simulink model "tb_drive_foc"  (R2026b)
settings: Solver=ode3  StopTime=1  FixedStep=P.drive.Ts_foc_plant  EnableMultiTasking=on
model workspace (MAT data in the model file):
  tb_J = 1.2798
  tb_Rsrc = 0.02
  tb_T_amb = 318.15
  tb_Trr = 6.97491
  tb_cmd.enable = timeseries
  tb_cmd.enable.Name = 'unnamed'
  tb_cmd.enable.DataInfo = tsdata.datametadata
  tb_cmd.enable.DataInfo.Interpolation = tsdata.interpolation
  tb_cmd.enable.DataInfo.Interpolation.Fhandle : function handle (value not decoded)
  tb_cmd.enable.DataInfo.Interpolation.Name = 'linear'
  tb_cmd.enable.TimeInfo = tsdata.timemetadata
  tb_cmd.enable.TimeInfo.Length = 1
  tb_cmd.enable.TimeInfo.DuplicateTimes = 0
  tb_cmd.enable.TimeInfo.Time_ = 0
  tb_cmd.enable.TimeInfo.Initialized = 1
  tb_cmd.enable.QualityInfo = tsdata.qualmetadata
  tb_cmd.enable.Data_ = 0
  tb_cmd.mode = timeseries
  tb_cmd.mode.Name = 'unnamed'
  tb_cmd.mode.DataInfo = tsdata.datametadata
  tb_cmd.mode.DataInfo.Interpolation = tsdata.interpolation
  tb_cmd.mode.DataInfo.Interpolation.Fhandle : function handle (value not decoded)
  tb_cmd.mode.DataInfo.Interpolation.Name = 'linear'
  tb_cmd.mode.TimeInfo = tsdata.timemetadata
  tb_cmd.mode.TimeInfo.Length = 1
  tb_cmd.mode.TimeInfo.DuplicateTimes = 0
  tb_cmd.mode.TimeInfo.Time_ = 0
  tb_cmd.mode.TimeInfo.Initialized = 1
  tb_cmd.mode.QualityInfo = tsdata.qualmetadata
  tb_cmd.mode.Data_ = 1
  tb_cmd.w_ref = timeseries
  tb_cmd.w_ref.Name = 'unnamed'
  tb_cmd.w_ref.DataInfo = tsdata.datametadata
  tb_cmd.w_ref.DataInfo.Interpolation = tsdata.interpolation
  tb_cmd.w_ref.DataInfo.Interpolation.Fhandle : function handle (value not decoded)
  tb_cmd.w_ref.DataInfo.Interpolation.Name = 'linear'
  tb_cmd.w_ref.TimeInfo = tsdata.timemetadata
  tb_cmd.w_ref.TimeInfo.Length = 1
  tb_cmd.w_ref.TimeInfo.DuplicateTimes = 0
  tb_cmd.w_ref.TimeInfo.Time_ = 0
  tb_cmd.w_ref.TimeInfo.Initialized = 1
  tb_cmd.w_ref.QualityInfo = tsdata.qualmetadata
  tb_cmd.w_ref.Data_ = 0
  tb_cmd.tau_ff = timeseries
  tb_cmd.tau_ff.Name = 'unnamed'
  tb_cmd.tau_ff.DataInfo = tsdata.datametadata
  tb_cmd.tau_ff.DataInfo.Interpolation = tsdata.interpolation
  tb_cmd.tau_ff.DataInfo.Interpolation.Fhandle : function handle (value not decoded)
  tb_cmd.tau_ff.DataInfo.Interpolation.Name = 'linear'
  tb_cmd.tau_ff.TimeInfo = tsdata.timemetadata
  tb_cmd.tau_ff.TimeInfo.Length = 1
  tb_cmd.tau_ff.TimeInfo.DuplicateTimes = 0
  tb_cmd.tau_ff.TimeInfo.Time_ = 0
  tb_cmd.tau_ff.TimeInfo.Initialized = 1
  tb_cmd.tau_ff.QualityInfo = tsdata.qualmetadata
  tb_cmd.tau_ff.Data_ = 0
  tb_cmd.tau_lim_mot = timeseries
  tb_cmd.tau_lim_mot.Name = 'unnamed'
  tb_cmd.tau_lim_mot.DataInfo = tsdata.datametadata
  tb_cmd.tau_lim_mot.DataInfo.Interpolation = tsdata.interpolation
  tb_cmd.tau_lim_mot.DataInfo.Interpolation.Fhandle : function handle (value not decoded)
  tb_cmd.tau_lim_mot.DataInfo.Interpolation.Name = 'linear'
  tb_cmd.tau_lim_mot.TimeInfo = tsdata.timemetadata
  tb_cmd.tau_lim_mot.TimeInfo.Length = 1
  tb_cmd.tau_lim_mot.TimeInfo.DuplicateTimes = 0
  tb_cmd.tau_lim_mot.TimeInfo.Time_ = 0
  tb_cmd.tau_lim_mot.TimeInfo.Initialized = 1
  tb_cmd.tau_lim_mot.QualityInfo = tsdata.qualmetadata
  tb_cmd.tau_lim_mot.Data_ = 16
  tb_cmd.tau_lim_reg = timeseries
  tb_cmd.tau_lim_reg.Name = 'unnamed'
  tb_cmd.tau_lim_reg.DataInfo = tsdata.datametadata
  tb_cmd.tau_lim_reg.DataInfo.Interpolation = tsdata.interpolation
  tb_cmd.tau_lim_reg.DataInfo.Interpolation.Fhandle : function handle (value not decoded)
  tb_cmd.tau_lim_reg.DataInfo.Interpolation.Name = 'linear'
  tb_cmd.tau_lim_reg.TimeInfo = tsdata.timemetadata
  tb_cmd.tau_lim_reg.TimeInfo.Length = 1
  tb_cmd.tau_lim_reg.TimeInfo.DuplicateTimes = 0
  tb_cmd.tau_lim_reg.TimeInfo.Time_ = 0
  tb_cmd.tau_lim_reg.TimeInfo.Initialized = 1
  tb_cmd.tau_lim_reg.QualityInfo = tsdata.qualmetadata
  tb_cmd.tau_lim_reg.Data_ = 16
  tb_cmd.park_req = timeseries
  tb_cmd.park_req.Name = 'unnamed'
  tb_cmd.park_req.DataInfo = tsdata.datametadata
  tb_cmd.park_req.DataInfo.Interpolation = tsdata.interpolation
  tb_cmd.park_req.DataInfo.Interpolation.Fhandle : function handle (value not decoded)
  tb_cmd.park_req.DataInfo.Interpolation.Name = 'linear'
  tb_cmd.park_req.TimeInfo = tsdata.timemetadata
  tb_cmd.park_req.TimeInfo.Length = 1
  tb_cmd.park_req.TimeInfo.DuplicateTimes = 0
  tb_cmd.park_req.TimeInfo.Time_ = 0
  tb_cmd.park_req.TimeInfo.Initialized = 1
  tb_cmd.park_req.QualityInfo = tsdata.qualmetadata
  tb_cmd.park_req.Data_ = 0
  tb_cmd.fault_reset = timeseries
  tb_cmd.fault_reset.Name = 'unnamed'
  tb_cmd.fault_reset.DataInfo = tsdata.datametadata
  tb_cmd.fault_reset.DataInfo.Interpolation = tsdata.interpolation
  tb_cmd.fault_reset.DataInfo.Interpolation.Fhandle : function handle (value not decoded)
  tb_cmd.fault_reset.DataInfo.Interpolation.Name = 'linear'
  tb_cmd.fault_reset.TimeInfo = tsdata.timemetadata
  tb_cmd.fault_reset.TimeInfo.Length = 1
  tb_cmd.fault_reset.TimeInfo.DuplicateTimes = 0
  tb_cmd.fault_reset.TimeInfo.Time_ = 0
  tb_cmd.fault_reset.TimeInfo.Initialized = 1
  tb_cmd.fault_reset.QualityInfo = tsdata.qualmetadata
  tb_cmd.fault_reset.Data_ = 0
  tb_cmd.alive = timeseries
  tb_cmd.alive.Name = 'unnamed'
  tb_cmd.alive.DataInfo = tsdata.datametadata
  tb_cmd.alive.DataInfo.Interpolation = tsdata.interpolation
  tb_cmd.alive.DataInfo.Interpolation.Fhandle : function handle (value not decoded)
  tb_cmd.alive.DataInfo.Interpolation.Name = 'linear'
  tb_cmd.alive.TimeInfo = tsdata.timemetadata
  tb_cmd.alive.TimeInfo.Length = 1
  tb_cmd.alive.TimeInfo.DuplicateTimes = 0
  tb_cmd.alive.TimeInfo.Time_ = 0
  tb_cmd.alive.TimeInfo.Initialized = 1
  tb_cmd.alive.QualityInfo = tsdata.qualmetadata
  tb_cmd.alive.Data_ = 0
  tb_contactor = timeseries
  tb_contactor.Name = 'unnamed'
  tb_contactor.DataInfo = tsdata.datametadata
  tb_contactor.DataInfo.Interpolation = tsdata.interpolation
  tb_contactor.DataInfo.Interpolation.Fhandle : function handle (value not decoded)
  tb_contactor.DataInfo.Interpolation.Name = 'linear'
  tb_contactor.TimeInfo = tsdata.timemetadata
  tb_contactor.TimeInfo.Length = 1
  tb_contactor.TimeInfo.DuplicateTimes = 0
  tb_contactor.TimeInfo.Time_ = 0
  tb_contactor.TimeInfo.Initialized = 1
  tb_contactor.QualityInfo = tsdata.qualmetadata
  tb_contactor.Data_ = 1
  tb_dec = 1
  tb_drop = timeseries
  tb_drop.Name = 'unnamed'
  tb_drop.DataInfo = tsdata.datametadata
  tb_drop.DataInfo.Interpolation = tsdata.interpolation
  tb_drop.DataInfo.Interpolation.Fhandle : function handle (value not decoded)
  tb_drop.DataInfo.Interpolation.Name = 'linear'
  tb_drop.TimeInfo = tsdata.timemetadata
  tb_drop.TimeInfo.Length = 1
  tb_drop.TimeInfo.DuplicateTimes = 0
  tb_drop.TimeInfo.Time_ = 0
  tb_drop.TimeInfo.Initialized = 1
  tb_drop.QualityInfo = tsdata.qualmetadata
  tb_drop.Data_ = 0
  tb_fi.L.can_drop = timeseries
  tb_fi.L.can_drop.Name = 'unnamed'
  tb_fi.L.can_drop.DataInfo = tsdata.datametadata
  tb_fi.L.can_drop.DataInfo.Interpolation = tsdata.interpolation
  tb_fi.L.can_drop.DataInfo.Interpolation.Fhandle : function handle (value not decoded)
  tb_fi.L.can_drop.DataInfo.Interpolation.Name = 'linear'
  tb_fi.L.can_drop.TimeInfo = tsdata.timemetadata
  tb_fi.L.can_drop.TimeInfo.Length = 1
  tb_fi.L.can_drop.TimeInfo.DuplicateTimes = 0
  tb_fi.L.can_drop.TimeInfo.Time_ = 0
  tb_fi.L.can_drop.TimeInfo.Initialized = 1
  tb_fi.L.can_drop.QualityInfo = tsdata.qualmetadata
  tb_fi.L.can_drop.Data_ = 0
  tb_fi.L.enc_fail = timeseries
  tb_fi.L.enc_fail.Name = 'unnamed'
  tb_fi.L.enc_fail.DataInfo = tsdata.datametadata
  tb_fi.L.enc_fail.DataInfo.Interpolation = tsdata.interpolation
  tb_fi.L.enc_fail.DataInfo.Interpolation.Fhandle : function handle (value not decoded)
  tb_fi.L.enc_fail.DataInfo.Interpolation.Name = 'linear'
  tb_fi.L.enc_fail.TimeInfo = tsdata.timemetadata
  tb_fi.L.enc_fail.TimeInfo.Length = 1
  tb_fi.L.enc_fail.TimeInfo.DuplicateTimes = 0
  tb_fi.L.enc_fail.TimeInfo.Time_ = 0
  tb_fi.L.enc_fail.TimeInfo.Initialized = 1
  tb_fi.L.enc_fail.QualityInfo = tsdata.qualmetadata
  tb_fi.L.enc_fail.Data_ = 0
  tb_fi.L.brake_stuck = timeseries
  tb_fi.L.brake_stuck.Name = 'unnamed'
  tb_fi.L.brake_stuck.DataInfo = tsdata.datametadata
  tb_fi.L.brake_stuck.DataInfo.Interpolation = tsdata.interpolation
  tb_fi.L.brake_stuck.DataInfo.Interpolation.Fhandle : function handle (value not decoded)
  tb_fi.L.brake_stuck.DataInfo.Interpolation.Name = 'linear'
  tb_fi.L.brake_stuck.TimeInfo = tsdata.timemetadata
  tb_fi.L.brake_stuck.TimeInfo.Length = 1
  tb_fi.L.brake_stuck.TimeInfo.DuplicateTimes = 0
  tb_fi.L.brake_stuck.TimeInfo.Time_ = 0
  tb_fi.L.brake_stuck.TimeInfo.Initialized = 1
  tb_fi.L.brake_stuck.QualityInfo = tsdata.qualmetadata
  tb_fi.L.brake_stuck.Data_ = 0
  tb_fi.L.tau_scale = timeseries
  tb_fi.L.tau_scale.Name = 'unnamed'
  tb_fi.L.tau_scale.DataInfo = tsdata.datametadata
  tb_fi.L.tau_scale.DataInfo.Interpolation = tsdata.interpolation
  tb_fi.L.tau_scale.DataInfo.Interpolation.Fhandle : function handle (value not decoded)
  tb_fi.L.tau_scale.DataInfo.Interpolation.Name = 'linear'
  tb_fi.L.tau_scale.TimeInfo = tsdata.timemetadata
  tb_fi.L.tau_scale.TimeInfo.Length = 1
  tb_fi.L.tau_scale.TimeInfo.DuplicateTimes = 0
  tb_fi.L.tau_scale.TimeInfo.Time_ = 0
  tb_fi.L.tau_scale.TimeInfo.Initialized = 1
  tb_fi.L.tau_scale.QualityInfo = tsdata.qualmetadata
  tb_fi.L.tau_scale.Data_ = 1
  tb_fi.L.T_offset = timeseries
  tb_fi.L.T_offset.Name = 'unnamed'
  tb_fi.L.T_offset.DataInfo = tsdata.datametadata
  tb_fi.L.T_offset.DataInfo.Interpolation = tsdata.interpolation
  tb_fi.L.T_offset.DataInfo.Interpolation.Fhandle : function handle (value not decoded)
  tb_fi.L.T_offset.DataInfo.Interpolation.Name = 'linear'
  tb_fi.L.T_offset.TimeInfo = tsdata.timemetadata
  tb_fi.L.T_offset.TimeInfo.Length = 1
  tb_fi.L.T_offset.TimeInfo.DuplicateTimes = 0
  tb_fi.L.T_offset.TimeInfo.Time_ = 0
  tb_fi.L.T_offset.TimeInfo.Initialized = 1
  tb_fi.L.T_offset.QualityInfo = tsdata.qualmetadata
  tb_fi.L.T_offset.Data_ = 0
  tb_fi.R.can_drop = timeseries
  tb_fi.R.can_drop.Name = 'unnamed'
  tb_fi.R.can_drop.DataInfo = tsdata.datametadata
  tb_fi.R.can_drop.DataInfo.Interpolation = tsdata.interpolation
  tb_fi.R.can_drop.DataInfo.Interpolation.Fhandle : function handle (value not decoded)
  tb_fi.R.can_drop.DataInfo.Interpolation.Name = 'linear'
  tb_fi.R.can_drop.TimeInfo = tsdata.timemetadata
  tb_fi.R.can_drop.TimeInfo.Length = 1
  tb_fi.R.can_drop.TimeInfo.DuplicateTimes = 0
  tb_fi.R.can_drop.TimeInfo.Time_ = 0
  tb_fi.R.can_drop.TimeInfo.Initialized = 1
  tb_fi.R.can_drop.QualityInfo = tsdata.qualmetadata
  tb_fi.R.can_drop.Data_ = 0
  tb_fi.R.enc_fail = timeseries
  tb_fi.R.enc_fail.Name = 'unnamed'
  tb_fi.R.enc_fail.DataInfo = tsdata.datametadata
  tb_fi.R.enc_fail.DataInfo.Interpolation = tsdata.interpolation
  tb_fi.R.enc_fail.DataInfo.Interpolation.Fhandle : function handle (value not decoded)
  tb_fi.R.enc_fail.DataInfo.Interpolation.Name = 'linear'
  tb_fi.R.enc_fail.TimeInfo = tsdata.timemetadata
  tb_fi.R.enc_fail.TimeInfo.Length = 1
  tb_fi.R.enc_fail.TimeInfo.DuplicateTimes = 0
  tb_fi.R.enc_fail.TimeInfo.Time_ = 0
  tb_fi.R.enc_fail.TimeInfo.Initialized = 1
  tb_fi.R.enc_fail.QualityInfo = tsdata.qualmetadata
  tb_fi.R.enc_fail.Data_ = 0
  tb_fi.R.brake_stuck = timeseries
  tb_fi.R.brake_stuck.Name = 'unnamed'
  tb_fi.R.brake_stuck.DataInfo = tsdata.datametadata
  tb_fi.R.brake_stuck.DataInfo.Interpolation = tsdata.interpolation
  tb_fi.R.brake_stuck.DataInfo.Interpolation.Fhandle : function handle (value not decoded)
  tb_fi.R.brake_stuck.DataInfo.Interpolation.Name = 'linear'
  tb_fi.R.brake_stuck.TimeInfo = tsdata.timemetadata
  tb_fi.R.brake_stuck.TimeInfo.Length = 1
  tb_fi.R.brake_stuck.TimeInfo.DuplicateTimes = 0
  tb_fi.R.brake_stuck.TimeInfo.Time_ = 0
  tb_fi.R.brake_stuck.TimeInfo.Initialized = 1
  tb_fi.R.brake_stuck.QualityInfo = tsdata.qualmetadata
  tb_fi.R.brake_stuck.Data_ = 0
  tb_fi.R.tau_scale = timeseries
  tb_fi.R.tau_scale.Name = 'unnamed'
  tb_fi.R.tau_scale.DataInfo = tsdata.datametadata
  tb_fi.R.tau_scale.DataInfo.Interpolation = tsdata.interpolation
  tb_fi.R.tau_scale.DataInfo.Interpolation.Fhandle : function handle (value not decoded)
  tb_fi.R.tau_scale.DataInfo.Interpolation.Name = 'linear'
  tb_fi.R.tau_scale.TimeInfo = tsdata.timemetadata
  tb_fi.R.tau_scale.TimeInfo.Length = 1
  tb_fi.R.tau_scale.TimeInfo.DuplicateTimes = 0
  tb_fi.R.tau_scale.TimeInfo.Time_ = 0
  tb_fi.R.tau_scale.TimeInfo.Initialized = 1
  tb_fi.R.tau_scale.QualityInfo = tsdata.qualmetadata
  tb_fi.R.tau_scale.Data_ = 1
  tb_fi.R.T_offset = timeseries
  tb_fi.R.T_offset.Name = 'unnamed'
  tb_fi.R.T_offset.DataInfo = tsdata.datametadata
  tb_fi.R.T_offset.DataInfo.Interpolation = tsdata.interpolation
  tb_fi.R.T_offset.DataInfo.Interpolation.Fhandle : function handle (value not decoded)
  tb_fi.R.T_offset.DataInfo.Interpolation.Name = 'linear'
  tb_fi.R.T_offset.TimeInfo = tsdata.timemetadata
  tb_fi.R.T_offset.TimeInfo.Length = 1
  tb_fi.R.T_offset.TimeInfo.DuplicateTimes = 0
  tb_fi.R.T_offset.TimeInfo.Time_ = 0
  tb_fi.R.T_offset.TimeInfo.Initialized = 1
  tb_fi.R.T_offset.QualityInfo = tsdata.qualmetadata
  tb_fi.R.T_offset.Data_ = 0
  tb_grade = timeseries
  tb_grade.Name = 'unnamed'
  tb_grade.DataInfo = tsdata.datametadata
  tb_grade.DataInfo.Interpolation = tsdata.interpolation
  tb_grade.DataInfo.Interpolation.Fhandle : function handle (value not decoded)
  tb_grade.DataInfo.Interpolation.Name = 'linear'
  tb_grade.TimeInfo = tsdata.timemetadata
  tb_grade.TimeInfo.Length = 1
  tb_grade.TimeInfo.DuplicateTimes = 0
  tb_grade.TimeInfo.Time_ = 0
  tb_grade.TimeInfo.Initialized = 1
  tb_grade.QualityInfo = tsdata.qualmetadata
  tb_grade.Data_ = 0
  tb_load = 1
  tb_sto = timeseries
  tb_sto.Name = 'unnamed'
  tb_sto.DataInfo = tsdata.datametadata
  tb_sto.DataInfo.Interpolation = tsdata.interpolation
  tb_sto.DataInfo.Interpolation.Fhandle : function handle (value not decoded)
  tb_sto.DataInfo.Interpolation.Name = 'linear'
  tb_sto.TimeInfo = tsdata.timemetadata
  tb_sto.TimeInfo.Length = 1
  tb_sto.TimeInfo.DuplicateTimes = 0
  tb_sto.TimeInfo.Time_ = 0
  tb_sto.TimeInfo.Initialized = 1
  tb_sto.QualityInfo = tsdata.qualmetadata
  tb_sto.Data_ = 1
  tb_vsrc = timeseries
  tb_vsrc.Name = 'unnamed'
  tb_vsrc.DataInfo = tsdata.datametadata
  tb_vsrc.DataInfo.Interpolation = tsdata.interpolation
  tb_vsrc.DataInfo.Interpolation.Fhandle : function handle (value not decoded)
  tb_vsrc.DataInfo.Interpolation.Name = 'linear'
  tb_vsrc.TimeInfo = tsdata.timemetadata
  tb_vsrc.TimeInfo.Length = 1
  tb_vsrc.TimeInfo.DuplicateTimes = 0
  tb_vsrc.TimeInfo.Time_ = 0
  tb_vsrc.TimeInfo.Initialized = 1
  tb_vsrc.QualityInfo = tsdata.qualmetadata
  tb_vsrc.Data_ = 46.8
  tb_w_dyno = timeseries
  tb_w_dyno.Name = 'unnamed'
  tb_w_dyno.DataInfo = tsdata.datametadata
  tb_w_dyno.DataInfo.Interpolation = tsdata.interpolation
  tb_w_dyno.DataInfo.Interpolation.Fhandle : function handle (value not decoded)
  tb_w_dyno.DataInfo.Interpolation.Name = 'linear'
  tb_w_dyno.TimeInfo = tsdata.timemetadata
  tb_w_dyno.TimeInfo.Length = 1
  tb_w_dyno.TimeInfo.DuplicateTimes = 0
  tb_w_dyno.TimeInfo.Time_ = 0
  tb_w_dyno.TimeInfo.Initialized = 1
  tb_w_dyno.QualityInfo = tsdata.qualmetadata
  tb_w_dyno.Data_ = 0
values from neighbouring files (symbols this model uses):
  P = evalin('base', 'P')    [build_tb_drive.m]    (also in tb_drive_long.m; tb_drive_profile.m)
undefined symbols (not defined in the file or in its folder): DiscIntNeverNeededParam
libraries: fl_lib x10, nesl_utility x5, simulink x1
settings Model: Creator=aomar  LastModifiedBy=aomar
settings ConfigSet: Description=Shaddad fixed-step 1 ms ode3, multitasking, explicit rate transitions (arch 7, D58).
settings DataIOCC: SignalLogging=off
settings OptimizationCC: SimCompilerOptimization=on
settings DebuggingCC: AlgebraicLoopMsg=error  ArtificialAlgebraicLoopMsg=error  SingleTaskRateTransMsg=error  StrictBusMsg=ErrorOnBusTreatedAsVector
settings SimscapeCC: SimscapeNominalValues="[{\"value\":\"1\",\"unit\":\"A\"},{\"value\":\"1\",\"unit\":\"bar\"},{\"value\":\"1\",\"unit\":\"cm^2\"},{\"value\":\"1\",\"unit\":\"cm^3/s\"},{\"value\":\"1\",\"unit\":\"kJ/kg\"},{\"value\":\"1\",\"unit\":\"kW\"},{\"value\":\"1\",\"unit\":\"l\"},{\"value\":\"1\",\"unit\":\"N\"},{\"value\":\"1\",\"unit\":\"N*m\"},{\"value\":\"1\",\"unit\":\"V\"},{\"value\":\"0.001\",\"unit\":\"Wb\"}]"  SimscapeNormalizeSystem=off  SimscapeUseEnergyAccounting=off

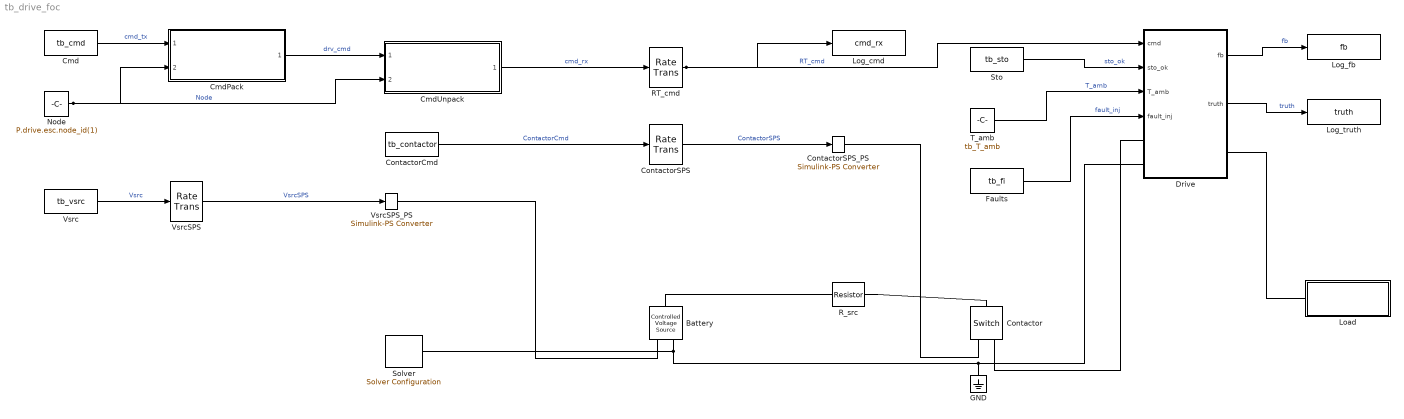
== system tb_drive_foc ==
  Battery : fl_lib/Electrical/Electrical Sources/Controlled Voltage Source
  Cmd : FromWorkspace  VariableName=tb_cmd  OutDataTypeStr=Bus: Bus_DriveSideCmd  SampleTime=P.drive.Ts_can  Interpolate=off  OutputAfterFinalValue=Holding final value
  CmdPack : Subsystem  ReferencedSubsystem=drive_cmd_pack
  CmdUnpack : Subsystem  ReferencedSubsystem=drive_cmd_unpack
  Contactor : fl_lib/Electrical/Electrical Elements/Switch  R_closed=1e-4 Ohm  G_open=1e-8 1/Ohm  Threshold=0.5  i_specify=off  i_priority=None  i=0 A  i_nominal_specify=off  i_nominal_value=1  i_nominal_unit=A  v_specify=off  v_priority=None  v=0 V  v_nominal_specify=off  v_nominal_value=1  v_nominal_unit=V
  ContactorCmd : FromWorkspace  VariableName=tb_contactor  SampleTime=P.drive.Ts_esc  Interpolate=off  OutputAfterFinalValue=Holding final value
  ContactorSPS : RateTransition  OutPortSampleTimeOpt=Inherit
  ContactorSPS_PS : nesl_utility/Simulink-PS Converter  PhysicalDomain=network_engine_domain  SubClassName=ps_input  LeftPortType=input  RightPortType=output  PseudoPeriodic=off  Frequencies=[]  NoiseDistribution=none  NoiseParameters=[]  Unit=1  AffineConversion=off  FilteringAndDerivatives=zero  SimscapeFilterOrder=1  InputFilterTimeConstant=0.001  UdotUserProvided=0
  Drive : Subsystem  mask{side=1}
  Faults : FromWorkspace  VariableName=tb_fi  OutDataTypeStr=Bus: Bus_DriveFaultInj  SampleTime=P.drive.Ts_esc  Interpolate=off  OutputAfterFinalValue=Holding final value
  GND : fl_lib/Electrical/Electrical Elements/Electrical Reference
  Load : Subsystem  Variant=on
  Log_cmd : ToWorkspace  VariableName=cmd_rx  SaveFormat=Timeseries  SampleTime=-1
      settings: Decimation=tb_dec
  Log_fb : ToWorkspace  VariableName=fb  SaveFormat=Timeseries  SampleTime=-1
      settings: Decimation=tb_dec
  Log_truth : ToWorkspace  VariableName=truth  SaveFormat=Timeseries  SampleTime=-1
      settings: Decimation=tb_dec
  Node : Constant  Value=P.drive.esc.node_id(1)  OutDataTypeStr=uint8
  RT_cmd : RateTransition  OutPortSampleTime=P.drive.Ts_esc
  R_src : fl_lib/Electrical/Electrical Elements/Resistor  R=tb_Rsrc Ohm  i_specify=off  i_priority=None  i=0 A  i_nominal_specify=off  i_nominal_value=1  i_nominal_unit=A  v_specify=off  v_priority=None  v=0 V  v_nominal_specify=off  v_nominal_value=1  v_nominal_unit=V
  Solver : nesl_utility/Solver Configuration  PhysicalDomain=network_engine_domain  SubClassName=solver  LeftPortType=input  RightPortType=generic  Tones=[]  Harmonics=[]  SimulateNoise=off  Profile=off  UseLocalSampling=off  EnableSwitchedLinearOptims=on  FrequencyDomain=off  UseCCode=off  RelTol=0.001  AbsTol=0.001  MinStep=1e-09  ToWorkspace=off  RevertToSquareIcSolve=off  NumHomotopyIterations=100  PhasorMode=off  PhasorModeNumHarmonics=1  ConsistencySolver=NEWTON_XTOL_AFTER_FTOL  CanonicalOrdering=CANONICAL  OptimizeIntermediates=OPTIMIZED  MulticoreSolverChoice=BACKWARD_EULER  IndexReductionMethod=DerivativeReplacement  DoDC=off  ResidualTolerance=1e-09  ConsistencyTolSource=GLOBAL  ConsistencyAbsTol=0.001  ConsistencyRelTol=0.001  ConsistencyTolFactor=0.001  UseLocalSolver=on  LocalSolverChoice=NE_BACKWARD_EULER_ADVANCER  ResolveIndetEquations=on  FunctionEvalNumThread=1  LocalSolverSampleTime=P.drive.Ts_foc_plant  DoFixedCost=on  MaxNonlinIter=P.sim.ssc.MaxNonlinIter  MaxModeIter=P.sim.ssc.MaxModeIter  ComputeImpulses=off  ImpulseIterations=2  LinearAlgebra=auto  LinearAlgebraNumThread=0  EquationFormulation=NE_TIME_EF  DelaysMemoryBudget=1024  AutomaticFiltering=on  FilteringTimeConstant=0.001  PartitionStorageMethod=AS_NEEDED  PartitionMemoryBudget=1024  PartitionMethod=BALANCED  MultibodyUseLocalSolver=off  MultibodyLocalSolverChoice=ODE1  MultibodyLocalSolverSampleTime=0.001
  Sto : FromWorkspace  VariableName=tb_sto  OutDataTypeStr=boolean  SampleTime=P.drive.Ts_esc  Interpolate=off  OutputAfterFinalValue=Holding final value
  T_amb : Constant  Value=tb_T_amb  SampleTime=P.drive.Ts_esc
  Vsrc : FromWorkspace  VariableName=tb_vsrc  SampleTime=P.drive.Ts_esc  Interpolate=off  OutputAfterFinalValue=Holding final value
  VsrcSPS : RateTransition  OutPortSampleTimeOpt=Inherit
  VsrcSPS_PS : nesl_utility/Simulink-PS Converter  PhysicalDomain=network_engine_domain  SubClassName=ps_input  LeftPortType=input  RightPortType=output  PseudoPeriodic=off  Frequencies=[]  NoiseDistribution=none  NoiseParameters=[]  Unit=V  AffineConversion=off  FilteringAndDerivatives=zero  SimscapeFilterOrder=1  InputFilterTimeConstant=0.001  UdotUserProvided=0
  wires:
  Node/1 -> CmdPack/2, CmdUnpack/2  "Node"
  Cmd/1 -> CmdPack/1  "cmd_tx"
  Vsrc/1 -> VsrcSPS/1  "Vsrc"
  VsrcSPS/1 -> VsrcSPS_PS/1  "VsrcSPS"
  CmdPack/1 -> CmdUnpack/1  "drv_cmd"
  ContactorCmd/1 -> ContactorSPS/1  "ContactorCmd"
  CmdUnpack/1 -> RT_cmd/1  "cmd_rx"
  RT_cmd/1 -> Log_cmd/1, Drive/1(cmd)  "RT_cmd"
  ContactorSPS/1 -> ContactorSPS_PS/1  "ContactorSPS"
  T_amb/1 -> Drive/3(T_amb)  "T_amb"
  Sto/1 -> Drive/2(sto_ok)  "sto_ok"
  Faults/1 -> Drive/4(fault_inj)  "fault_inj"
  Drive/1(fb) -> Log_fb/1  "fb"
  Drive/2(truth) -> Log_truth/1  "truth"
  connections:
  Battery/LConn1 -- R_src/LConn1
  VsrcSPS_PS/RConn1 -- Battery/RConn1
  R_src/RConn1 -- Contactor/LConn1
  Drive/LConn1 -- Contactor/RConn2
  Drive/RConn1 -- Load/LConn1
  Battery/RConn2 -- Solver/RConn1 -- GND/LConn1 -- Drive/LConn2
  ContactorSPS_PS/RConn1 -- Contactor/RConn1

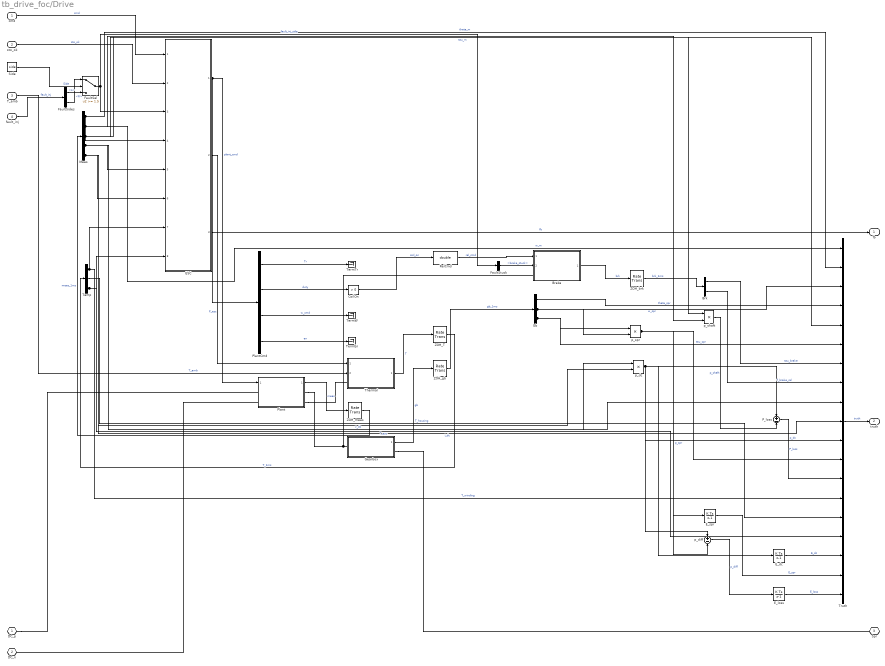
== system tb_drive_foc/Drive ==
  cmd : Inport  OutDataTypeStr=Bus: Bus_DriveSideCmd  SampleTime=P.drive.Ts_esc
  sto_ok : Inport  Port=2  OutDataTypeStr=boolean  SampleTime=P.drive.Ts_esc
  T_amb : Inport  Port=3  OutDataTypeStr=double  SampleTime=P.drive.Ts_esc
  fault_inj : Inport  Port=4  OutDataTypeStr=Bus: Bus_DriveFaultInj  SampleTime=P.drive.Ts_esc
  Brake : Subsystem  ReferencedSubsystem=drive_brake
  Brk : Demux  Outputs=2
  CoilOn : simulink/Logic and Bit Operations/Compare To Constant  relop=>  const=0  OutDataTypeStr=boolean
  ESC : Subsystem  ReferencedSubsystem=drive_esc
  E_dc : DiscreteIntegrator  gainval=1  SampleTime=P.drive.Ts_esc  ICPrevOutput=DiscIntNeverNeededParam  ICPrevScaledInput=DiscIntNeverNeededParam
  E_loss : DiscreteIntegrator  gainval=1  SampleTime=P.drive.Ts_esc  ICPrevOutput=DiscIntNeverNeededParam  ICPrevScaledInput=DiscIntNeverNeededParam
  E_spr : DiscreteIntegrator  gainval=1  SampleTime=P.drive.Ts_esc  ICPrevOutput=DiscIntNeverNeededParam  ICPrevScaledInput=DiscIntNeverNeededParam
  FaultSel : Switch  Threshold=1.5  SaturateOnIntegerOverflow=off  InputSameDT=off
  FaultSides : BusSelector  OutputSignals=L,R
  FaultStuck : BusSelector  OutputSignals=brake_stuck
  Gb : Demux  Outputs=3
  Gearbox : Subsystem  ReferencedSubsystem=drive_gearbox
  Meas : Demux  Outputs=5
  P_loss : Sum  Inputs=+-
  Plant : Subsystem  ReferencedSubsystem=drive_plant_foc
  PlantCmd : Demux
  RelCmd : DataTypeConversion  OutDataTypeStr=double  RndMeth=Nearest
  Side : Constant  Value=side
  Temp : Demux  Outputs=3
  TermEn : Terminator
  TermTr : Terminator
  TermW : Terminator
  Thermal : Subsystem  ReferencedSubsystem=drive_thermal
  Truth : BusCreator  Inputs=19  OutDataTypeStr=Bus: Bus_DriveSideTruth  NonVirtualBus=on
  ZOH_T : RateTransition  OutPortSampleTime=P.drive.Ts_esc
  ZOH_brk : RateTransition  OutPortSampleTime=P.drive.Ts_esc
  ZOH_gb : RateTransition  OutPortSampleTime=P.drive.Ts_esc
  ZOH_meas : RateTransition  OutPortSampleTime=P.drive.Ts_esc
  p_dc : Product  Inputs=**
  p_diff : Sum  Inputs=+-
  p_shaft : Product  Inputs=**
  p_spr : Product  Inputs=**
  DC_p : PMIOPort  Side=Left  ConnectionType=Connection: foundation.electrical.electrical
  DC_n : PMIOPort  Port=2  Side=Left  ConnectionType=Connection: foundation.electrical.electrical
  Spr : PMIOPort  Port=3  Side=Right  ConnectionType=Connection: foundation.mechanical.rotational.rotational
  fb : Outport  OutDataTypeStr=Bus: Bus_DriveSideFb
  truth : Outport  Port=2  OutDataTypeStr=Bus: Bus_DriveSideTruth
  wires:
  cmd/1 -> ESC/1  "cmd"
  sto_ok/1 -> ESC/2  "sto_ok"
  Side/1 -> FaultSel/2  "Side"
  T_amb/1 -> Thermal/2  "T_amb"
  fault_inj/1 -> FaultSides/1  "fault_inj"
  FaultSides/1 -> FaultSel/3  "<L>"
  FaultSides/2 -> FaultSel/1  "<R>"
  Meas/1 -> Truth/2, ESC/4  "theta_m"
  Meas/2 -> p_shaft/2, Truth/1  "w_m"
  Meas/3 -> Truth/5, p_shaft/1  "tau_m"
  Meas/4 -> Truth/9, p_dc/1, ESC/5  "v_dc"
  Meas/5 -> Truth/10, p_dc/2, ESC/6  "i_dc"
  Temp/1 -> Truth/14, ESC/7  "T_winding"
  Temp/2 -> Truth/15  "T_housing"
  Temp/3 -> Truth/16, ESC/8  "T_esc"
  FaultSel/1 -> FaultStuck/1, ESC/3  "fault_inj_side"
  ESC/1 -> Plant/1, PlantCmd/1  "plant_cmd"
  ESC/2 -> Thermal/1  "P_esc"
  ESC/3 -> fb/1  "fb"
  PlantCmd/1 -> TermTr/1  "Tr"
  PlantCmd/2 -> CoilOn/1  "duty"
  PlantCmd/3 -> TermW/1  "w_cmd"
  PlantCmd/4 -> TermEn/1  "en"
  Plant/1 -> ZOH_meas/1  "meas"
  CoilOn/1 -> RelCmd/1  "coil_on"
  ZOH_meas/1 -> Meas/1  "meas_1ms"
  Thermal/1 -> ZOH_T/1  "T"
  Gearbox/1 -> ZOH_gb/1  "gb"
  ZOH_T/1 -> Temp/1  "T_1ms"
  ZOH_gb/1 -> Gb/1  "gb_1ms"
  RelCmd/1 -> Brake/1  "rel_cmd"
  FaultStuck/1 -> Brake/2  "<brake_stuck>"
  Gb/1 -> Truth/4  "theta_spr"
  Gb/2 -> p_spr/2, Truth/3  "w_spr"
  Gb/3 -> Truth/6, p_spr/1  "tau_spr"
  Brake/1 -> ZOH_brk/1  "brk"
  p_spr/1 -> p_diff/2, E_spr/1, Truth/12  "p_spr"
  ZOH_brk/1 -> Brk/1  "brk_1ms"
  p_dc/1 -> E_dc/1, p_diff/1, Truth/11, P_loss/1  "p_dc"
  Brk/1 -> Truth/7  "tau_brake"
  Brk/2 -> Truth/8  "f_brake_rel"
  p_diff/1 -> E_loss/1  "p_diff"
  p_shaft/1 -> P_loss/2  "p_shaft"
  E_spr/1 -> Truth/18  "E_spr"
  P_loss/1 -> Truth/13  "P_loss"
  E_dc/1 -> Truth/17  "E_dc"
  E_loss/1 -> Truth/19  "E_loss"
  Truth/1 -> truth/1  "truth"
  connections:
  Gearbox/LConn1 -- Plant/RConn1 -- Brake/LConn1
  Plant/LConn2 -- DC_n/RConn1
  DC_p/RConn1 -- Plant/LConn1
  Gearbox/RConn1 -- Spr/RConn1
  Plant/RConn2 -- Thermal/LConn1

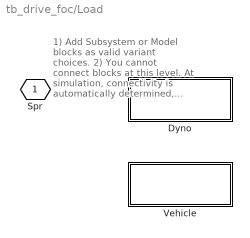
== system tb_drive_foc/Load ==
  note: 1) Add Subsystem or Model blocks as valid variant choices.
      | 2) You cannot connect blocks at this level. At simulation, connectivity is automatically
      | determined, based on the active variant and port name matching.
  Dyno : Subsystem  VariantControl=tb_load == 2
  Vehicle : Subsystem  VariantControl=tb_load == 1
  Spr : PMIOPort  Side=Left  ConnectionType=Connection: foundation.mechanical.rotational.rotational

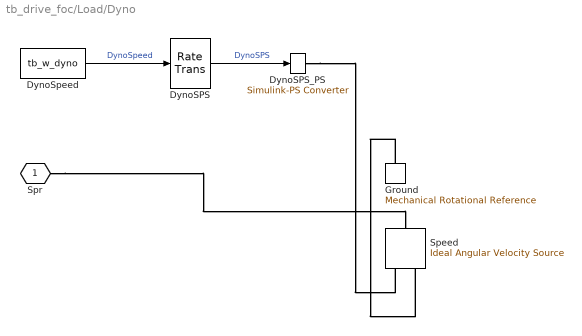
== system tb_drive_foc/Load/Dyno ==
  DynoSPS : RateTransition  OutPortSampleTimeOpt=Inherit
  DynoSPS_PS : nesl_utility/Simulink-PS Converter  PhysicalDomain=network_engine_domain  SubClassName=ps_input  LeftPortType=input  RightPortType=output  PseudoPeriodic=off  Frequencies=[]  NoiseDistribution=none  NoiseParameters=[]  Unit=rad/s  AffineConversion=off  FilteringAndDerivatives=zero  SimscapeFilterOrder=1  InputFilterTimeConstant=0.001  UdotUserProvided=0
  DynoSpeed : FromWorkspace  VariableName=tb_w_dyno  SampleTime=P.drive.Ts_esc  Interpolate=off  OutputAfterFinalValue=Holding final value
  Ground : fl_lib/Mechanical/Rotational Elements/Mechanical Rotational Reference
  Speed : fl_lib/Mechanical/Mechanical Sources/Ideal Angular Velocity Source
  Spr : PMIOPort  Side=Left  ConnectionType=Connection: foundation.mechanical.rotational.rotational
  wires:
  DynoSpeed/1 -> DynoSPS/1  "DynoSpeed"
  DynoSPS/1 -> DynoSPS_PS/1  "DynoSPS"
  connections:
  DynoSPS_PS/RConn1 -- Speed/RConn1
  Ground/LConn1 -- Speed/RConn2
  Spr/RConn1 -- Speed/LConn1

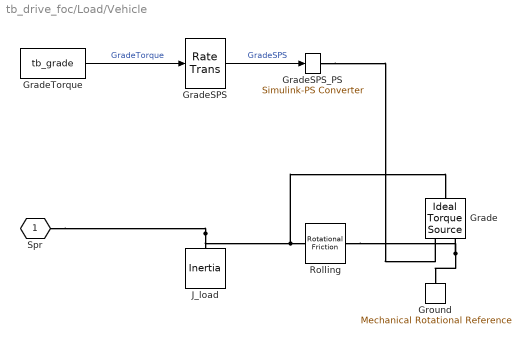
== system tb_drive_foc/Load/Vehicle ==
  Grade : fl_lib/Mechanical/Mechanical Sources/Ideal Torque Source
  GradeSPS : RateTransition  OutPortSampleTimeOpt=Inherit
  GradeSPS_PS : nesl_utility/Simulink-PS Converter  PhysicalDomain=network_engine_domain  SubClassName=ps_input  LeftPortType=input  RightPortType=output  PseudoPeriodic=off  Frequencies=[]  NoiseDistribution=none  NoiseParameters=[]  Unit=N*m  AffineConversion=off  FilteringAndDerivatives=zero  SimscapeFilterOrder=1  InputFilterTimeConstant=0.001  UdotUserProvided=0
  GradeTorque : FromWorkspace  VariableName=tb_grade  SampleTime=P.drive.Ts_esc  Interpolate=off  OutputAfterFinalValue=Holding final value
  Ground : fl_lib/Mechanical/Rotational Elements/Mechanical Rotational Reference
  J_load : fl_lib/Mechanical/Rotational Elements/Inertia  inertia=tb_J kg*m^2  num_ports=foundation.enum.numPorts2.one  w_specify=off  w_priority=High  w=0 rad/s  w_nominal_specify=off  w_nominal_value=1  w_nominal_unit=rad/s  t_specify=off  t_priority=None  t=0 N*m  t_nominal_specify=off  t_nominal_value=1  t_nominal_unit=N*m
  Rolling : fl_lib/Mechanical/Rotational Elements/Rotational Friction  brkwy_trq=1.0001*tb_Trr N*m  brkwy_vel=P.drive.bench.w_brk_rr rad/s  Col_trq=tb_Trr N*m  visc_coef=0 N*m*s/rad  w_specify=off  w_priority=None  w=0 rad/s  w_nominal_specify=off  w_nominal_value=1  w_nominal_unit=rad/s  t_specify=off  t_priority=None  t=0 N*m  t_nominal_specify=off  t_nominal_value=1  t_nominal_unit=N*m
  Spr : PMIOPort  Side=Left  ConnectionType=Connection: foundation.mechanical.rotational.rotational
  wires:
  GradeTorque/1 -> GradeSPS/1  "GradeTorque"
  GradeSPS/1 -> GradeSPS_PS/1  "GradeSPS"
  connections:
  J_load/LConn1 -- Spr/RConn1 -- Rolling/LConn1 -- Grade/LConn1
  GradeSPS_PS/RConn1 -- Grade/RConn1
  Grade/RConn2 -- Rolling/RConn1 -- Ground/LConn1
